simulink model "ThreePhaseFullyControlledConverter"  (R2024b)
settings: Solver=VariableStepAuto  StartTime=0.0  StopTime=10  RelTol=1e-3
undefined symbols (not defined in the file): a
libraries: spsThyristorLib x6, spsSeriesRLCBranchLib x1, spsThreePhaseVIMeasurementLib x1, spsThreePhaseSourceLib x1, spsVoltageMeasurementLib x1, sps_lib x1
settings Model: Creator=lenovo  LastModifiedBy=lenovo

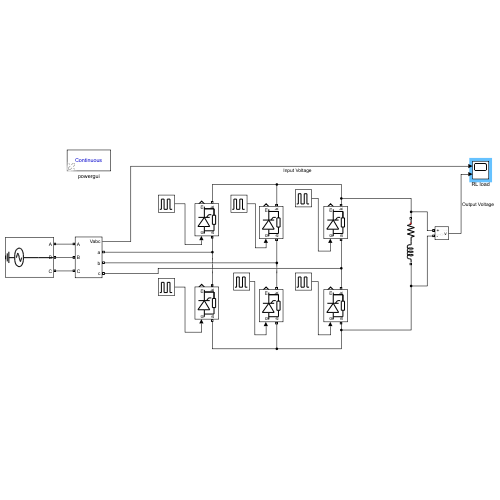
[thumbnail: Simulink's stored preview of the top-level diagram]
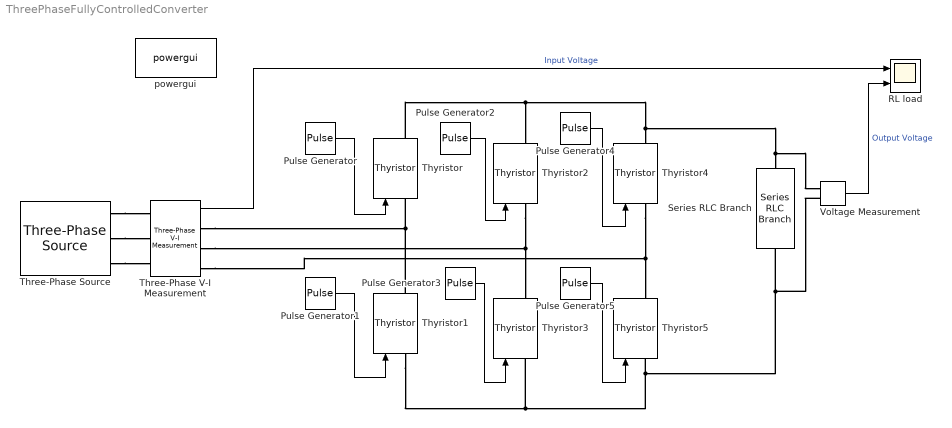
== system ThreePhaseFullyControlledConverter ==
  Pulse Generator : DiscretePulseGenerator  PulseType=Time based  Period=0.02  PulseWidth=10  PhaseDelay=a*0.02/360
  Pulse Generator1 : DiscretePulseGenerator  PulseType=Time based  Period=0.02  PulseWidth=10  PhaseDelay=(a+180)*0.02/360
  Pulse Generator2 : DiscretePulseGenerator  PulseType=Time based  Period=0.02  PulseWidth=10  PhaseDelay=(a+120)*0.02/360
  Pulse Generator3 : DiscretePulseGenerator  PulseType=Time based  Period=0.02  PulseWidth=10  PhaseDelay=(a+300)*0.02/360
  Pulse Generator4 : DiscretePulseGenerator  PulseType=Time based  Period=0.02  PulseWidth=10  PhaseDelay=(a+240)*0.02/360
  Pulse Generator5 : DiscretePulseGenerator  PulseType=Time based  Period=0.02  PulseWidth=10  PhaseDelay=(a+60)*0.02/360
  RL load : Scope  NumInputPorts=2
  Series RLC Branch : spsSeriesRLCBranchLib/Series RLC Branch  LConnTagsString=__new0  RConnTagsString=__new0  BranchType=RL  Resistance=1000  Inductance=25e-3  SetiL0=off  InitialCurrent=0  Capacitance=1e-6  Setx0=off  InitialVoltage=0  Measurements=None
  Three-Phase V-I Measurement : spsThreePhaseVIMeasurementLib/Three-Phase V-I Measurement  VoltageMeasurement=phase-to-ground  SetLabelV=off  LabelV=Vabc  Vpu=off  VpuLL=off  CurrentMeasurement=no  SetLabelI=off  LabelI=Iabc  Ipu=off  Pbase=100e6  Vbase=500e3  OutputType=Complex  PhasorSimulation=off  PSBequivalent=0
  Three-Phase Source : spsThreePhaseSourceLib/Three-Phase Source  InternalConnection=Yg  VoltagePhases=off  Voltage=25e3  PhaseAngle=0  Voltage_phases=[25e3 25e3 25e3]/sqrt(3)  PhaseAngles_phases=[0 -120 +120]  Frequency=60  NonIdealSource=on  SpecifyImpedance=off  Resistance=0  Inductance=0  ShortCircuitLevel=100e6  BaseVoltage=25e3  XRratio=7  BusType=swing  Pref=10e3  Qref=0  Prefabc=[10e3, 10e3, 10e3]  Qrefabc=[0, 0, 0]  Qmin=-inf  Qmax=inf
  Thyristor{,1..5} (6 alike) : spsThyristorLib/Thyristor  Ron=0.001  Lon=0  Vf=0.8  IC=0  Rs=500  Cs=250e-9  Measurements=on
  Voltage Measurement : spsVoltageMeasurementLib/Voltage Measurement  PhasorSimulation=off  OutputType=Complex  PSBequivalent=0
  powergui : sps_lib/powergui  Priority=1  SimulationMode=Continuous  SampleTime=50e-6  frequency=60  Iterations=50  frequencyindice=60  Pbase=100e6  ErrMax=1e-4  UnitsV=kV  UnitsW=MW  buscounter=0  FunctionMessages=off  echomessages=off  EnableUseOfTLC=off  CurrentSourceSwitches=off  DisableSnubberDevices=off  DisableRonSwitches=off  DisableVfSwitches=off  DisplayEquations=off  AutomaticDiscreteSolvers=off  SolverType=Tustin/Backward Euler (TBE)  Interpol=off  ExternalGateDelay=off  methode=off  Ts=100  x0status=blocks  SPID=on  SwTol=0  HookPort=off  NonlinearTolerance=1e-4  nMaxIteration=100  ContinueOnMaxIteration=off  RestoreLinks=warning  ResistiveCurrentMeasurement=off  Frange=[0:2:500]  Ylog=off  Xlog=on  ShowGrid=off  save=off  variable=ZData  structure=0  ZoomFFT=off  StartTime=0.0  cycles=1  DisplayStyle=1  fundamental=60  FreqAxis=off  MaxFrequency=1000  frequencyindicesteady=1  RmsSteady=1  display=off
  wires:
  Three-Phase V-I Measurement/1 -> RL load/1  "Input Voltage"
  Voltage Measurement/1 -> RL load/2  "Output Voltage"
  Pulse Generator/1 -> Thyristor/1
  Pulse Generator1/1 -> Thyristor1/1
  Pulse Generator2/1 -> Thyristor2/1
  Pulse Generator3/1 -> Thyristor3/1
  Pulse Generator4/1 -> Thyristor4/1
  Pulse Generator5/1 -> Thyristor5/1
  connections:
  Three-Phase Source/RConn2 -- Three-Phase V-I Measurement/LConn2
  Three-Phase Source/RConn1 -- Three-Phase V-I Measurement/LConn1
  Three-Phase Source/RConn3 -- Three-Phase V-I Measurement/LConn3
  Thyristor1/RConn1 -- Thyristor/LConn1 -- Three-Phase V-I Measurement/RConn1
  Thyristor2/LConn1 -- Three-Phase V-I Measurement/RConn2 -- Thyristor3/RConn1
  Thyristor4/LConn1 -- Thyristor5/RConn1 -- Three-Phase V-I Measurement/RConn3
  Thyristor/RConn1 -- Voltage Measurement/LConn1 -- Series RLC Branch/LConn1 -- Thyristor4/RConn1 -- Thyristor2/RConn1
  Thyristor1/LConn1 -- Thyristor3/LConn1 -- Voltage Measurement/LConn2 -- Series RLC Branch/RConn1 -- Thyristor5/LConn1
